simulink model "sm_trackV_lib_belt_lower_frame_s45i2u0l3_ptcld"  (R2026b)
settings: Solver=VariableStepAuto
undefined symbols (not defined in the file): Fixed, Left, Trac, track_seg_tgts_seg45i2u0r3, X, Y, Z
libraries: sm_trackV_lib_belt_contact x2, sm_lib x2, sm_trackV_lib_belt_track_s45 x1, sm_trackV_lib_belt_underc_idlerArm_i2u0l3 x1
settings Model: Creator=smiller  LastModifiedBy=smiller

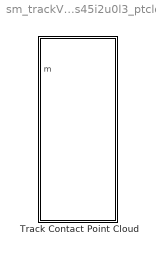
== system sm_trackV_lib_belt_lower_frame_s45i2u0l3_ptcld ==
  Track Contact Point Cloud : Subsystem  VariantControl=BeltPts  mask(Lower Frame Belted Track, Two Idler, Point Cloud){sprk_wid_roll=Trac.Sprocket.Roller.wid, sprk_rad_roll=Trac.Sprocket.Roller.rad, sprk_clr=Trac.Sprocket.Roller.clr, sprk_opc=Trac.Sprocket.Roller.opc, sprk_rad_pitch=Trac.Sprocket.Spoke.pitch_rad, sprk_spoke_rad=Trac.Sprocket.Spoke.rad, sprk_spoke_num=Trac.Sprocket.nSpokes, sprk_spoke_len=Trac.Sprocket.Spoke.len, sprk_rim_spoke_xc=Trac.Sprocket.Rim.spoke_xc, sprk_rim_ir=Trac.Sprocket.Rim.rad_inner, sprk_rim_thk=Trac.Sprocket.Rim.thk, sprk_contgeo_roller_clr=Trac.Sprocket.roller_contact.clr, sprk_contgeo_roller_opc=Trac.Sprocket.roller_contact.opc, sprk_contgeo_spoke_clr=Trac.Sprocket.spoke_contact.clr, sprk_contgeo_spoke_opc=Trac.Sprocket.spoke_contact.opc, idlerR_rad=Trac.IdlerR.rad, idlerF_rad=Trac.IdlerF.rad, idlerR_len=Trac.IdlerR.len, idlerF_len=Trac.IdlerF.len, idlerR_wheel_clr=Trac.IdlerR.Wheel.clr, idlerF_wheel_clr=Trac.IdlerF.Wheel.clr, idlerR_rim_rad=Trac.IdlerR.Rim.rad, idlerF_rim_rad=Trac.IdlerF.Rim.rad, idlerR_rim_hub_rad=Trac.IdlerR.Rim.hub_rad, idlerF_rim_hub_rad=Trac.IdlerF.Rim.hub_rad, idlerR_rim_xc=Trac.IdlerR.Rim.rim_xc, idlerF_rim_xc=Trac.IdlerF.Rim.rim_xc, idlerR_rho=Trac.IdlerR.rho, idlerF_rho=Trac.IdlerF.rho, idlerR_clr=Trac.IdlerR.clr, idlerF_clr=Trac.IdlerF.clr, idlerR_opc=Trac.IdlerR.opc, idlerF_opc=Trac.IdlerF.opc, idlerR_axle_rad=Trac.IdlerR.Axle.rad, idlerF_axle_rad=Trac.IdlerF.Axle.rad, idlerR_axle_len=Trac.IdlerR.Axle.len, idlerF_axle_len=Trac.IdlerF.Axle.len, idlerR_axle_rho=Trac.IdlerR.Axle.rho, idlerF_axle_rho=Trac.IdlerF.Axle.rho, idlerR_axle_clr=Trac.IdlerR.Axle.clr, idlerF_axle_clr=Trac.IdlerF.Axle.clr, idlerR_axle_opc=Trac.IdlerR.Axle.opc, idlerF_axle_opc=Trac.IdlerF.Axle.opc, idlerR_contgeo_clr=Trac.IdlerR.belt_contact.clr, idlerF_contgeo_clr=Trac.IdlerF.belt_contact.clr, idlerR_contgeo_opc=Trac.IdlerR.belt_contact.opc, idlerF_contgeo_opc=Trac.IdlerF.belt_contact.opc, arm_idlerc=Trac.IdlerArm.Pivot_to_Idler, arm_tens_x=Trac.IdlerArm.Pivot_to_TensionerX, arm_tens_y=Trac.IdlerArm.Pivot_to_TensionerY, arm_wid=Trac.IdlerArm.wid, arm_thk=Trac.IdlerArm.thk, arm_rho=Trac.IdlerArm.rho, arm_clr=Trac.IdlerArm.clr, arm_opc=Trac.IdlerArm.opc, roller_lower_rad=Trac.Roller.Lower.rad, roller_lower_len=Trac.Roller.Lower.len, roller_lower_rho=Trac.Roller.Lower.rho, roller_lower_clr=Trac.Roller.Lower.clr, roller_lower_opc=Trac.Roller.Lower.opc, roller_lower_rim_thk=Trac.Roller.Lower.rim_thk, roller_lower_rim_len=Trac.Roller.Lower.rim_len, roller_lower_axle_rad=Trac.Roller.Lower.Axle.rad, roller_lower_axle_len=Trac.Roller.Lower.Axle.len, roller_lower_axle_rho=Trac.Roller.Lower.Axle.rho, roller_lower_axle_clr=Trac.Roller.Lower.Axle.clr, roller_lower_axle_opc=Trac.Roller.Lower.Axle.opc, roller_lower_contgeo_clr=Trac.Roller.Lower.belt_contact.clr, roller_lower_contgeo_opc=Trac.Roller.Lower.belt_contact.opc, tensioner_cyl_len=Trac.IdlerF.Tensioner.cyl.len, tensioner_cyl_rad=Trac.IdlerF.Tensioner.cyl.rad, tensioner_cyl_rho=Trac.IdlerF.Tensioner.cyl.rho, tensioner_cyl_clr=Trac.IdlerF.Tensioner.cyl.clr, tensioner_cyl_opc=Trac.IdlerF.Tensioner.cyl.opc, tensioner_pist_len=Trac.IdlerF.Tensioner.piston.len, tensioner_pist_rad=Trac.IdlerF.Tensioner.piston.rad, tensioner_pist_rho=Trac.IdlerF.Tensioner.piston.rho, tensioner_pist_clr=Trac.IdlerF.Tensioner.piston.clr, tensioner_pist_opc=Trac.IdlerF.Tensioner.piston.opc, tensioner_br_len=Trac.IdlerF.Tensioner.bracket.len, tensioner_br_width=Trac.IdlerF.Tensioner.bracket.wid, tensioner_br_height=Trac.IdlerF.Tensioner.bracket.height, tensioner_br_thk=Trac.IdlerF.Tensioner.bracket.thk, tensioner_br_rho=Trac.IdlerF.Tensioner.bracket.rho, tensioner_br_clr=Trac.IdlerF.Tensioner.bracket.clr, tensioner_br_opc=Trac.IdlerF.Tensioner.bracket.opc, tensioner_eqpos=Trac.IdlerF.Tensioner.xeq, tensioner_x0=Trac.IdlerF.Tensioner.x0, tensioner_k=Trac.IdlerF.Tensioner.K, tensioner_b=Trac.IdlerF.Tensioner.B, popup_leftOrRight=Left, popup_trackFrame=Fixed, roller_lower_x=Trac.Frame.SprkOffLon.Lower, idlerFix_x=Trac.Frame.SprkOffLon.IdlerR, idlerArm_x=Trac.Frame.SprkOffLon.IdlerArm, tensionC_x=Trac.Frame.SprkOffLon.TensionC, frame_pivot_x=Trac.Frame.SprkOffLon.PivotFra, axle_x=Trac.Frame.SprkOffLon.Axle, roller_lower_y=Trac.Frame.SprkOffVer.Lower, idlerFix_y=Trac.Frame.SprkOffVer.IdlerR, tensionC_y=Trac.Frame.SprkOffVer.TensionC, frame_pivot_y=Trac.Frame.SprkOffVer.PivotFra, axle_y=Trac.Frame.SprkOffVer.Axle, idlerArm_y=Trac.Frame.SprkOffVer.IdlerArm, frame_mass=Trac.Frame.TrackFrame.Mass, frame_cg_offset=Trac.Frame.TrackFrame.CG, frame_moi=Trac.Frame.TrackFrame.MOI, frame_poi=Trac.Frame.TrackFrame.POI, frame_roller_cg_offset=Trac.Frame.SprkFrame.CG, frame_roller_mass=Trac.Frame.SprkFrame.Mass, frame_roller_moi=Trac.Frame.SprkFrame.MOI, frame_roller_poi=Trac.Frame.SprkFrame.POI, frame_susp_offset=Trac.Frame.SuspOffset, roller_frame_pivot_range=Trac.Frame.PivotFra.Range, roller_frame_pivot_k=Trac.Frame.PivotFra.LimitK, roller_frame_pivot_b=Trac.Frame.PivotFra.LimitB, roller_frame_pivot_tw=Trac.Frame.PivotFra.LimitTW, carc_len=Trac.Belt.l, carc_wid=Trac.Belt.w, carc_thk=Trac.Belt.pad_h, carc_mass=Trac.Belt.mass, carc_cg=Trac.Belt.cg, carc_moi=Trac.Belt.moi, carc_poi=Trac.Belt.poi, carc_clr=Trac.Belt.clr, carc_opc=Trac.Belt.opc, lug_hei=Trac.Belt.Lug.h, lug_lb=Trac.Belt.Lug.lb, lug_lt=Trac.Belt.Lug.lt, lug_w=Trac.Belt.Lug.w, lug_xc=Trac.Belt.Lug.xc, lug_clr=Trac.Belt.clr, lug_opc=Trac.Belt.opc, jointTargets=track_seg_tgts_seg45i2u0r3, trackDamping=Trac.Belt.damping, lug_line_clr=Trac.Belt.lug_contact.clr, lug_line_opc=Trac.Belt.lug_contact.opc, carc_line_clr=Trac.Belt.carcass_contact.clr, carc_line_opc=Trac.Belt.carcass_contact.opc, ptcld_belt=Trac.Belt.ground_contact.ptcld.pts, ptcld_belt_rad=Trac.Belt.ground_contact.ptcld.rad, ptcld_belt_clr=Trac.Belt.ground_contact.ptcld.clr, ptcld_belt_opc=Trac.Belt.ground_contact.ptcld.opc, K_SprocketLug=Trac.Contact.SprocketLug.K, B_SprocketLug=Trac.Contact.SprocketLug.B, TW_SprocketLug=Trac.Contact.SprocketLug.TW, K_SprocketRoller=Trac.Contact.SprocketRoller.K, B_SprocketRoller=Trac.Contact.SprocketRoller.B, TW_SprocketRoller=Trac.Contact.SprocketRoller.TW, K_IdlerFix=Trac.Contact.IdlerR.K, B_IdlerFix=Trac.Contact.IdlerR.B, TW_IdlerFix=Trac.Contact.IdlerR.TW, K_IdlerArm=Trac.Contact.IdlerF.K, B_IdlerArm=Trac.Contact.IdlerF.B, TW_IdlerArm=Trac.Contact.IdlerF.TW, K_Roller=Trac.Contact.Roller.K, B_Roller=Trac.Contact.Roller.B, TW_Roller=Trac.Contact.Roller.TW, popup_sense_roller=Actuator Torque}
      mask prompts: sprk_wid_roll "Roller Width (m)"; sprk_rad_roll "Rolling Radius (m)"; sprk_clr "Color [R G B] (0-1)"; sprk_opc "Opacity (0-1)"; sprk_rad_pitch "Pitch Radius (m)"; sprk_spoke_rad "Radius (m)"; sprk_spoke_num "Number of Spokes"; sprk_spoke_len "Length (m)"; sprk_rim_spoke_xc "Spoke Cross Section [x y] (m)"; sprk_rim_ir "Inner Radius (m)"; sprk_rim_thk "Thickness (m)"; sprk_contgeo_roller_clr "Roller Color [R G B] (0-1)"; sprk_contgeo_roller_opc "Roller Opacity (0-1)"; sprk_contgeo_spoke_clr "Spoke Color [R G B] (0-1)"; sprk_contgeo_spoke_opc "Spoke Opacity (0-1)"; arm_idlerc "Offset Pivot to Idler Center (m)"; arm_tens_x "Offset Pivot to Tensioner Long. (m)"; arm_tens_y "Offset Pivot to Tensioner Vert. (m)"; arm_wid "Idler Arm Width (m)"; arm_thk "Idler Arm Thickness (m)"; arm_rho "Idler Arm Density"; arm_clr "Idler Arm Color [R G B] (m) (0-1)"; arm_opc "Opacity (0-1)"; roller_lower_rad "Radius (m)"; roller_lower_len "Length (m)"; roller_lower_rho "Density (kg/m^3)"; roller_lower_clr "Color [R G B] (0-1)"; roller_lower_opc "Opacity (0-1)"; roller_lower_rim_thk "Thickness (m)"; roller_lower_rim_len "Length (m)"; roller_lower_axle_rad "Radius (m)"; roller_lower_axle_len "Length (m)"; roller_lower_axle_rho "Density (kg/m^3)"; roller_lower_axle_clr "Color [R G B] (0-1)"; roller_lower_axle_opc "Opacity (0-1)"; roller_lower_contgeo_clr "Color [R G B] (0-1)"; roller_lower_contgeo_opc "Opacity (0-1)"; tensioner_cyl_len "Length (m)"; tensioner_cyl_rad "Radius (m)"; tensioner_cyl_rho "Density (kg/m^3)"; tensioner_cyl_clr "Color [R G B] (0-1)"; tensioner_cyl_opc "Opacity (0-1)"; tensioner_pist_len "Piston Length (m)"; tensioner_pist_rad "Radius (m)"; tensioner_pist_rho "Density (kg/m^3)"; tensioner_pist_clr "Color [R G B] (0-1)"; tensioner_pist_opc "Opacity (0.1)"; tensioner_br_len "Length (m)"; tensioner_br_width "Width (m)"; tensioner_br_height "Height (m)"; tensioner_br_thk "Bracket Thickness (m)"; tensioner_br_rho "Density (kg/m^3)"; tensioner_br_clr "Color [R G B] (0-1)"; tensioner_br_opc "Opacity (0.1)"; tensioner_eqpos "Equilibrium Position (m)"; tensioner_x0 "Assembly Position (m)"; tensioner_k "Stiffness Coefficient (N/m)"; tensioner_b "Damping Coefficient (N/(m/s))"; popup_leftOrRight "Left or Right"; popup_trackFrame "Track Frame"; roller_lower_x "Lower Rollers (vector) (m)"; idlerFix_x "Idler Wheel Fixed (m)"; idlerArm_x "Idler Arm (m)"; tensionC_x "Tensioner Cylinder (m)"; frame_pivot_x "Frame Pivot (m)"; axle_x "Axle (m)"; roller_lower_y "Lower Rollers (m)"; idlerFix_y "Idler Wheel Fixed (m)"; tensionC_y "Tensioner Cylinder (m)"; frame_pivot_y "Frame Pivot (m)"; axle_y "Axle (m)"; idlerArm_y "Idler Arm (m)"; frame_mass "Mass (kg)"; frame_cg_offset "CG Offset from Sprocket [x y z] (m)"; frame_moi "Moments of Inertia [Ixx Iyy Izz] (kg*m^2)"; frame_poi "Products of Inertia [Ixx Iyy Izz] (kg*m^2)"; frame_roller_cg_offset "CG Offset from Sprocket [x y z] (m)"; frame_roller_mass "Mass (kg)"; frame_roller_moi "Moments of Inertia [Ixx Iyy Izz] (kg*m^2)"; frame_roller_poi "Products of Inertia [Ixx Iyy Izz] (kg*m^2)"; frame_susp_offset "Suspension Offset from Sprocket [x y z] (m)"; roller_frame_pivot_range "Range (deg)"; roller_frame_pivot_k "Stop stiffness (N*m/deg)"; roller_frame_pivot_b "Stop damping (N*m/(deg*sec)"; roller_frame_pivot_tw "Stop transition width (deg)"; carc_len "Length (m)"; carc_wid "Width (m)"; carc_thk "Thickness (m)"; carc_mass "Mass (kg)"; carc_cg "CG [x y z] (kg)"; carc_moi "Moments of Inertia [Ixx Iyy Izz] (kg*m^2)"; carc_poi "Products of Inertia [Iyz Ixz Ixy] (kg*m^2)"; carc_clr "Color [R G B]"; carc_opc "Opacity (0-1)"; lug_hei "Height (m)"; lug_lb "Length Base (m)"; lug_lt "Length Tip (m)"; lug_w "Width (m)"; lug_xc "Profile [x y] (m)"; lug_clr "Color [R G B]"; lug_opc "Opacity (0-1)"; jointTargets "Joint Targets (structure)"; trackDamping "Joint Damping N*m/(deg/s)"; lug_line_clr "Color [R G B] (0-1)"; lug_line_opc "Opacity (0-1)"; carc_line_clr "Color [R G B] (0-1)"; carc_line_opc "Opacity (0-1)"; ptcld_belt "Points [x y z] (m)"; ptcld_belt_rad "Radius (m)"; ptcld_belt_clr "Color [R G B] (0-1)"; ptcld_belt_opc "Opacity (0-1)"; K_SprocketLug "Normal Stiffness (N/m)"; B_SprocketLug "Normal Damping (N/(m/s))"; TW_SprocketLug "Normal Transition Width (m)"; K_SprocketRoller "Normal Stiffness (N/m)"; B_SprocketRoller "Normal Damping (N/(m/s))"; TW_SprocketRoller "Normal Transition Width (m)"; K_IdlerFix "Normal Stiffness (N/m)"; B_IdlerFix "Normal Damping (N/(m/s))"; TW_IdlerFix "Normal Transition Width (m)"; K_IdlerArm "Normal Stiffness (N/m)"; B_IdlerArm "Normal Damping (N/(m/s))"; TW_IdlerArm "Normal Transition Width (m)"; K_Roller "Normal Stiffness (N/m)"; B_Roller "Normal Damping (N/(m/s))"; TW_Roller "Normal Transition Width (m)"; popup_sense_roller "Roller"
      mask help: Models a segmented belt with undercarriage. Contact geometry (point cloud) in belt segment enables contact with the ground. Includes sprocket, rollers, and idler with tensioner. The sprocket has a 1D rotational mechanical interface to the drivetrain.
      settings: AttributesFormatString=|
      | %<popup_leftOrRight>
      | %<popup_sense_roller>
      | %<popup_trackFrame>
      mask TypeOptions sprk_wid_roll: Undercarriage/sprk_wid_roll
      mask TypeOptions sprk_rad_roll: Undercarriage/sprk_rad_roll
      mask TypeOptions sprk_clr: Undercarriage/sprk_clr
      mask TypeOptions sprk_opc: Undercarriage/sprk_opc
      mask TypeOptions sprk_rad_pitch: Undercarriage/sprk_rad_pitch
      mask TypeOptions sprk_spoke_rad: Undercarriage/sprk_spoke_rad
      mask TypeOptions sprk_spoke_num: Undercarriage/sprk_spoke_num
      mask TypeOptions sprk_spoke_len: Undercarriage/sprk_spoke_len
      mask TypeOptions sprk_rim_spoke_xc: Undercarriage/sprk_rim_spoke_xc
      mask TypeOptions sprk_rim_ir: Undercarriage/sprk_rim_ir
      mask TypeOptions sprk_rim_thk: Undercarriage/sprk_rim_thk
      mask TypeOptions sprk_contgeo_roller_clr: Undercarriage/sprk_contgeo_roller_clr
      mask TypeOptions sprk_contgeo_roller_opc: Undercarriage/sprk_contgeo_roller_opc
      mask TypeOptions sprk_contgeo_spoke_clr: Undercarriage/sprk_contgeo_spoke_clr
      mask TypeOptions sprk_contgeo_spoke_opc: Undercarriage/sprk_contgeo_spoke_opc
      mask TypeOptions idlerR_rad: Undercarriage/idlerR_rad
      mask TypeOptions idlerF_rad: Undercarriage/idlerF_rad
      mask TypeOptions idlerR_len: Undercarriage/idlerR_len
      mask TypeOptions idlerF_len: Undercarriage/idlerF_len
      mask TypeOptions idlerR_wheel_clr: Undercarriage/idlerR_wheel_clr
      mask TypeOptions idlerF_wheel_clr: Undercarriage/idlerF_wheel_clr
      mask TypeOptions idlerR_rim_rad: Undercarriage/idlerR_rim_rad
      mask TypeOptions idlerF_rim_rad: Undercarriage/idlerF_rim_rad
      mask TypeOptions idlerR_rim_hub_rad: Undercarriage/idlerR_rim_hub_rad
      mask TypeOptions idlerF_rim_hub_rad: Undercarriage/idlerF_rim_hub_rad
      mask TypeOptions idlerR_rim_xc: Undercarriage/idlerR_rim_xc
      mask TypeOptions idlerF_rim_xc: Undercarriage/idlerF_rim_xc
      mask TypeOptions idlerR_rho: Undercarriage/idlerR_rho
      mask TypeOptions idlerF_rho: Undercarriage/idlerF_rho
      mask TypeOptions idlerR_clr: Undercarriage/idlerR_clr
      mask TypeOptions idlerF_clr: Undercarriage/idlerF_clr
      mask TypeOptions idlerR_opc: Undercarriage/idlerR_opc
      mask TypeOptions idlerF_opc: Undercarriage/idlerF_opc
      mask TypeOptions idlerR_axle_rad: Undercarriage/idlerR_axle_rad
      mask TypeOptions idlerF_axle_rad: Undercarriage/idlerF_axle_rad
      mask TypeOptions idlerR_axle_len: Undercarriage/idlerR_axle_len
      mask TypeOptions idlerF_axle_len: Undercarriage/idlerF_axle_len
      mask TypeOptions idlerR_axle_rho: Undercarriage/idlerR_axle_rho
      mask TypeOptions idlerF_axle_rho: Undercarriage/idlerF_axle_rho
      mask TypeOptions idlerR_axle_clr: Undercarriage/idlerR_axle_clr
      mask TypeOptions idlerF_axle_clr: Undercarriage/idlerF_axle_clr
      mask TypeOptions idlerR_axle_opc: Undercarriage/idlerR_axle_opc
      mask TypeOptions idlerF_axle_opc: Undercarriage/idlerF_axle_opc
      mask TypeOptions idlerR_contgeo_clr: Undercarriage/idlerR_contgeo_clr
      mask TypeOptions idlerF_contgeo_clr: Undercarriage/idlerF_contgeo_clr
      mask TypeOptions idlerR_contgeo_opc: Undercarriage/idlerR_contgeo_opc
      mask TypeOptions idlerF_contgeo_opc: Undercarriage/idlerF_contgeo_opc
      mask TypeOptions arm_idlerc: Undercarriage/arm_idlerc
      mask TypeOptions arm_tens_x: Undercarriage/arm_tens_x
      mask TypeOptions arm_tens_y: Undercarriage/arm_tens_y
      mask TypeOptions arm_wid: Undercarriage/arm_wid
      mask TypeOptions arm_thk: Undercarriage/arm_thk
      mask TypeOptions arm_rho: Undercarriage/arm_rho
      mask TypeOptions arm_clr: Undercarriage/arm_clr
      mask TypeOptions arm_opc: Undercarriage/arm_opc
      mask TypeOptions roller_lower_rad: Undercarriage/roller_lower_rad
      mask TypeOptions roller_lower_len: Undercarriage/roller_lower_len
      mask TypeOptions roller_lower_rho: Undercarriage/roller_lower_rho
      mask TypeOptions roller_lower_clr: Undercarriage/roller_lower_clr
      mask TypeOptions roller_lower_opc: Undercarriage/roller_lower_opc
      mask TypeOptions roller_lower_rim_thk: Undercarriage/roller_lower_rim_thk
      mask TypeOptions roller_lower_rim_len: Undercarriage/roller_lower_rim_len
      mask TypeOptions roller_lower_axle_rad: Undercarriage/roller_lower_axle_rad
      mask TypeOptions roller_lower_axle_len: Undercarriage/roller_lower_axle_len
      mask TypeOptions roller_lower_axle_rho: Undercarriage/roller_lower_axle_rho
      mask TypeOptions roller_lower_axle_clr: Undercarriage/roller_lower_axle_clr
      mask TypeOptions roller_lower_axle_opc: Undercarriage/roller_lower_axle_opc
      mask TypeOptions roller_lower_contgeo_clr: Undercarriage/roller_lower_contgeo_clr
      mask TypeOptions roller_lower_contgeo_opc: Undercarriage/roller_lower_contgeo_opc
      mask TypeOptions tensioner_cyl_len: Undercarriage/tensioner_cyl_len
      mask TypeOptions tensioner_cyl_rad: Undercarriage/tensioner_cyl_rad
      mask TypeOptions tensioner_cyl_rho: Undercarriage/tensioner_cyl_rho
      mask TypeOptions tensioner_cyl_clr: Undercarriage/tensioner_cyl_clr
      mask TypeOptions tensioner_cyl_opc: Undercarriage/tensioner_cyl_opc
      mask TypeOptions tensioner_pist_len: Undercarriage/tensioner_pist_len
      mask TypeOptions tensioner_pist_rad: Undercarriage/tensioner_pist_rad
      mask TypeOptions tensioner_pist_rho: Undercarriage/tensioner_pist_rho
      mask TypeOptions tensioner_pist_clr: Undercarriage/tensioner_pist_clr
      mask TypeOptions tensioner_pist_opc: Undercarriage/tensioner_pist_opc
      mask TypeOptions tensioner_br_len: Undercarriage/tensioner_br_len
      mask TypeOptions tensioner_br_width: Undercarriage/tensioner_br_width
      mask TypeOptions tensioner_br_height: Undercarriage/tensioner_br_height
      mask TypeOptions tensioner_br_thk: Undercarriage/tensioner_br_thk
      mask TypeOptions tensioner_br_rho: Undercarriage/tensioner_br_rho
      mask TypeOptions tensioner_br_clr: Undercarriage/tensioner_br_clr
      mask TypeOptions tensioner_br_opc: Undercarriage/tensioner_br_opc
      mask TypeOptions tensioner_eqpos: Undercarriage/tensioner_eqpos
      mask TypeOptions tensioner_x0: Undercarriage/tensioner_x0
      mask TypeOptions tensioner_k: Undercarriage/tensioner_k
      mask TypeOptions tensioner_b: Undercarriage/tensioner_b
      mask TypeOptions popup_leftOrRight: Undercarriage/popup_leftOrRight
      mask TypeOptions popup_trackFrame: Undercarriage/popup_trackFrame
      mask TypeOptions roller_lower_x: Undercarriage/roller_lower_x
      mask TypeOptions idlerFix_x: Undercarriage/idlerFix_x
      mask TypeOptions idlerArm_x: Undercarriage/idlerArm_x
      mask TypeOptions tensionC_x: Undercarriage/tensionC_x
      mask TypeOptions frame_pivot_x: Undercarriage/frame_pivot_x
      mask TypeOptions axle_x: Undercarriage/axle_x
      mask TypeOptions roller_lower_y: Undercarriage/roller_lower_y
      mask TypeOptions idlerFix_y: Undercarriage/idlerFix_y
      mask TypeOptions tensionC_y: Undercarriage/tensionC_y
      mask TypeOptions frame_pivot_y: Undercarriage/frame_pivot_y
      mask TypeOptions axle_y: Undercarriage/axle_y
      mask TypeOptions idlerArm_y: Undercarriage/idlerArm_y
      mask TypeOptions frame_mass: Undercarriage/frame_mass
      mask TypeOptions frame_cg_offset: Undercarriage/frame_cg_offset
      mask TypeOptions frame_moi: Undercarriage/frame_moi
      mask TypeOptions frame_poi: Undercarriage/frame_poi
      mask TypeOptions frame_roller_cg_offset: Undercarriage/frame_roller_cg_offset
      mask TypeOptions frame_roller_mass: Undercarriage/frame_roller_mass
      mask TypeOptions frame_roller_moi: Undercarriage/frame_roller_moi
      mask TypeOptions frame_roller_poi: Undercarriage/frame_roller_poi
      mask TypeOptions frame_susp_offset: Undercarriage/frame_susp_offset
      mask TypeOptions roller_frame_pivot_range: Undercarriage/roller_frame_pivot_range
      mask TypeOptions roller_frame_pivot_k: Undercarriage/roller_frame_pivot_k
      mask TypeOptions roller_frame_pivot_b: Undercarriage/roller_frame_pivot_b
      mask TypeOptions roller_frame_pivot_tw: Undercarriage/roller_frame_pivot_tw
      mask TypeOptions carc_len: Track/carc_len
      mask TypeOptions carc_wid: Track/carc_wid
      mask TypeOptions carc_thk: Track/carc_thk
      mask TypeOptions carc_mass: Track/carc_mass
      mask TypeOptions carc_cg: Track/carc_cg
      mask TypeOptions carc_moi: Track/carc_moi
      mask TypeOptions carc_poi: Track/carc_poi
      mask TypeOptions carc_clr: Track/carc_clr
      mask TypeOptions carc_opc: Track/carc_opc
      mask TypeOptions lug_hei: Track/lug_hei
      mask TypeOptions lug_lb: Track/lug_lb
      mask TypeOptions lug_lt: Track/lug_lt
      mask TypeOptions lug_w: Track/lug_w
      mask TypeOptions lug_xc: Track/lug_xc
      mask TypeOptions lug_clr: Track/lug_clr
      mask TypeOptions lug_opc: Track/lug_opc
      mask TypeOptions jointTargets: Track/jointTargets
      mask TypeOptions trackDamping: Track/trackDamping
      mask TypeOptions lug_line_clr: Track/lug_line_clr
      mask TypeOptions lug_line_opc: Track/lug_line_opc
      mask TypeOptions carc_line_clr: Track/carc_line_clr
      mask TypeOptions carc_line_opc: Track/carc_line_opc
      mask TypeOptions ptcld_belt: Track/ptcld_belt
      mask TypeOptions ptcld_belt_rad: Track/ptcld_belt_rad
      mask TypeOptions ptcld_belt_clr: Track/ptcld_belt_clr
      mask TypeOptions ptcld_belt_opc: Track/ptcld_belt_opc
      mask TypeOptions K_SprocketLug:
      | CF
      | Sprocket
      | Lugs/K_SprocketLug
      mask TypeOptions B_SprocketLug:
      | CF
      | Sprocket
      | Lugs/B_SprocketLug
      mask TypeOptions TW_SprocketLug:
      | CF
      | Sprocket
      | Lugs/TW_SprocketLug
      mask TypeOptions K_SprocketRoller:
      | CF
      | Belt
      | Roller/K_SprocketRoller
      mask TypeOptions B_SprocketRoller:
      | CF
      | Belt
      | Roller/B_SprocketRoller
      mask TypeOptions TW_SprocketRoller:
      | CF
      | Belt
      | Roller/TW_SprocketRoller
      mask TypeOptions K_IdlerFix:
      | CF
      | Belt
      | Roller/K_IdlerFix
      mask TypeOptions B_IdlerFix:
      | CF
      | Belt
      | Roller/B_IdlerFix
      mask TypeOptions TW_IdlerFix:
      | CF
      | Belt
      | Roller/TW_IdlerFix
      mask TypeOptions K_IdlerArm:
      | CF
      | Belt
      | Roller/K_IdlerArm
      mask TypeOptions B_IdlerArm:
      | CF
      | Belt
      | Roller/B_IdlerArm
      mask TypeOptions TW_IdlerArm:
      | CF
      | Belt
      | Roller/TW_IdlerArm
      mask TypeOptions K_Roller:
      | CF
      | Belt
      | Roller/K_Roller
      mask TypeOptions B_Roller:
      | CF
      | Belt
      | Roller/B_Roller
      mask TypeOptions TW_Roller:
      | CF
      | Belt
      | Roller/TW_Roller
      mask TypeOptions popup_sense_roller: Undercarriage/popup_sense_roller
      mask DialogControl cont_sprocket Prompt: Sprocket
      mask DialogControl cont_sprk_roller Prompt: Roller
      mask DialogControl cont_sprk_spoke Prompt: Spoke
      mask DialogControl cont_sprk_rim Prompt: Rim
      mask DialogControl cont_contgeo_sprk Prompt: Contact Geometry
      mask DialogControl cont_idler Prompt: Idler
      mask DialogControl cont_idler_roller Prompt: Roller
      mask DialogControl text_idler_rear Prompt: Rear
      mask DialogControl text_idler_front Prompt: Front
      mask DialogControl text_idler_rad Prompt: Radius (m)
      mask DialogControl text_idler_len Prompt: Length (m)
      mask DialogControl text_idler_wheel_clr Prompt: Wheel Color [R G B] (0-1)
      mask DialogControl cont_idler_rim Prompt: Rim
      mask DialogControl text_idler_rim_rad Prompt: Radius (m)
      mask DialogControl text_idler_hub_rad Prompt: Hub Radius (m)
      mask DialogControl text_idler_rim_xc Prompt: Cross Section [x y] (m)
      mask DialogControl text_idler_rho Prompt: Density (kg/m^3)
      mask DialogControl text_idler_clr Prompt: Color [R G B] (0-1)
      mask DialogControl text_idler_opc Prompt: Opacity (0-1)
      mask DialogControl cont_idler_axle Prompt: Axle
      mask DialogControl text_idler_axle_rad Prompt: Radius (m)
      mask DialogControl text_idler_axle_len Prompt: Length (m)
      mask DialogControl text_idler_axle_rho Prompt: Density (kg/m^3)
      mask DialogControl text_idler_axle_clr Prompt: Color [R G B] (0-1)
      mask DialogControl text_idler_axle_opc Prompt: Opacity (0-1)
      mask DialogControl cont_idler_pin_contgeo Prompt: Contact Geometry
      mask DialogControl text_idler_contgeo_clr Prompt: Color [R G B] (0-1)
      mask DialogControl text_idler_contgeo_opc Prompt: Opacity (0-1)
      mask DialogControl cont_idler_arm Prompt: Idler Arm
      mask DialogControl cont_roller_lower Prompt: Rollers
      mask DialogControl cont_rollerL_roller Prompt: Roller
      mask DialogControl cont_rollerL_rim Prompt: Rim
      mask DialogControl cont_rollerL_axle Prompt: Axle
      mask DialogControl cont_rollerL_contgeo Prompt: Contact Geometry
      mask DialogControl cont_tensioner Prompt: Tensioner
      mask DialogControl cont_tens_cyl Prompt: Cylinder
      mask DialogControl cont_tens_pist Prompt: Piston
      mask DialogControl cont_tens_brk Prompt: Bracket
      mask DialogControl cont_tens_asy Prompt: Assembly
      mask DialogControl cont_frame Prompt: Frame
      mask DialogControl cont_frame_lon Prompt: Longitudinal Offsets from Sprocket
      mask DialogControl cont_frame_ver Prompt: Vertical Offsets from Sprocket
      mask DialogControl cont_frame_mass Prompt: Mass and Inertia
      mask DialogControl cont_sprocket_frame Prompt: Sprocket Frame
      mask DialogControl cont_roller_frame Prompt: Roller Frame
      mask DialogControl cont_susp_offset Prompt: Suspension Offsets
      mask DialogControl cont_frame_pivot Prompt: Frame Pivot
      mask DialogControl cont_belt Prompt: Belt
      mask DialogControl cont_carcass Prompt: Carcass
      mask DialogControl cont_lug Prompt: Lug
      mask DialogControl cont_belt_assy Prompt: Assembly
      mask DialogControl cont_contgeo_belt Prompt: Contact Geometry
      mask DialogControl cont_contgeo_lug2sprk Prompt: Sprocket to Lug
      mask DialogControl cont_contgeo_carc2roll Prompt: Carcass to Rollers
      mask DialogControl cont_contgeo_carc2gnd Prompt: Carcass to Ground
      mask DialogControl cont_contact Prompt: Contact
      mask DialogControl cont_contact_lug2sprk Prompt: Lug to Sprocket
      mask DialogControl cont_contact_carc2sprk Prompt: Carcass to Sprocket Roller
      mask DialogControl cont_contact_carc2idlerX Prompt: Carcass to Fixed Idler
      mask DialogControl cont_contact_carc2idlerA Prompt: Carcass to Moving Idler
      mask DialogControl cont_contact_carc2roller Prompt: Carcass to Rollers
      mask DialogControl cont_sensing Prompt: Sensing
      mask Display: image('sm_belt_track_2i_ptcld_topview_IMAGE.png')

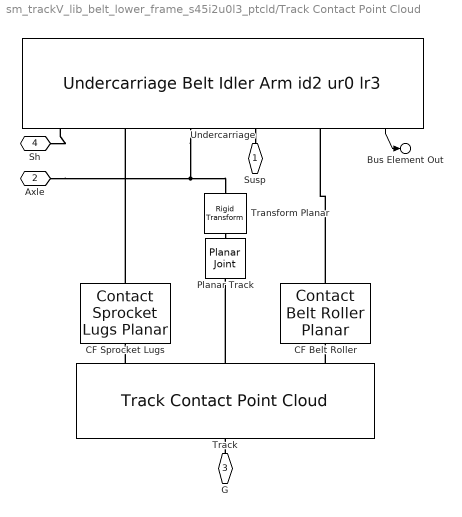
== system sm_trackV_lib_belt_lower_frame_s45i2u0l3_ptcld/Track Contact Point Cloud ==
  " CF Sprocket Lugs" : sm_trackV_lib_belt_contact/Contact Sprocket Lugs Planar  K_SprocketLug=K_SprocketLug  B_SprocketLug=B_SprocketLug  TW_SprocketLug=TW_SprocketLug
  CF Belt Roller : sm_trackV_lib_belt_contact/Contact Belt Roller Planar  K_SprocketRoller=K_SprocketRoller  B_SprocketRoller=B_SprocketRoller  TW_SprocketRoller=TW_SprocketRoller  K_IdlerFix=K_IdlerFix  B_IdlerFix=B_IdlerFix  TW_IdlerFix=TW_IdlerFix  K_IdlerArm=K_IdlerArm  B_IdlerArm=B_IdlerArm  TW_IdlerArm=TW_IdlerArm  K_Roller=K_Roller  B_Roller=B_Roller  TW_Roller=TW_Roller
  Planar Track : sm_lib/Joints/Planar Joint  JointMode=Normal  CompositeWrenchDir=FollowerOnBase  CompositeWrenchFrame=BaseFrame  SenseConstraintForce=off  SenseConstraintTorque=off  SenseTotalForce=off  SenseTotalTorque=off  PxPositionTargetSpecify=on  PxPositionTargetPriority=High  PxPositionTargetValue=0  PxPositionTargetValueUnits=m  PxVelocityTargetSpecify=off  PxVelocityTargetPriority=High  PxVelocityTargetValue=0  PxVelocityTargetValueUnits=m/s  PxEquilibriumPosition=0  PxEquilibriumPositionUnits=m  PxSpringStiffness=0  PxSpringStiffnessUnits=N/m  PxDampingCoefficient=0  PxDampingCoefficientUnits=N/(m/s)  PxLowerLimitSpecify=off  PxLowerLimitBound=-1  PxLowerLimitBoundUnits=m  PxLowerLimitStiffness=1e6  PxLowerLimitStiffnessUnits=N/m  PxLowerLimitDamping=1e3  PxLowerLimitDampingUnits=N/(m/s)  PxLowerLimitTransitionRegionWidth=1e-4  PxLowerLimitTransitionRegionWidthUnits=m  PxUpperLimitSpecify=off  PxUpperLimitBound=1  PxUpperLimitBoundUnits=m  PxUpperLimitStiffness=1e6  PxUpperLimitStiffnessUnits=N/m  PxUpperLimitDamping=1e3  PxUpperLimitDampingUnits=N/(m/s)  PxUpperLimitTransitionRegionWidth=1e-4  PxUpperLimitTransitionRegionWidthUnits=m  PxTorqueActuationMode=NoTorque  PxMotionActuationMode=ComputedMotion  PxSensePosition=off  PxSenseVelocity=off  PxSenseAcceleration=off  PxSenseTorqueForce=off  PxSenseLowerLimitTorqueForce=off  PxSenseUpperLimitTorqueForce=off  PyPositionTargetSpecify=on  PyPositionTargetPriority=High  PyPositionTargetValue=0  PyPositionTargetValueUnits=m  PyVelocityTargetSpecify=off  PyVelocityTargetPriority=High  PyVelocityTargetValue=0  PyVelocityTargetValueUnits=m/s  PyEquilibriumPosition=0  PyEquilibriumPositionUnits=m  PySpringStiffness=0  PySpringStiffnessUnits=N/m  PyDampingCoefficient=0  PyDampingCoefficientUnits=N/(m/s)  PyLowerLimitSpecify=off  PyLowerLimitBound=-1  PyLowerLimitBoundUnits=m  PyLowerLimitStiffness=1e6  PyLowerLimitStiffnessUnits=N/m  PyLowerLimitDamping=1e3  PyLowerLimitDampingUnits=N/(m/s)  PyLowerLimitTransitionRegionWidth=1e-4  PyLowerLimitTransitionRegionWidthUnits=m  PyUpperLimitSpecify=off  PyUpperLimitBound=1  PyUpperLimitBoundUnits=m  PyUpperLimitStiffness=1e6  PyUpperLimitStiffnessUnits=N/m  PyUpperLimitDamping=1e3  PyUpperLimitDampingUnits=N/(m/s)  PyUpperLimitTransitionRegionWidth=1e-4  PyUpperLimitTransitionRegionWidthUnits=m  PyTorqueActuationMode=NoTorque  PyMotionActuationMode=ComputedMotion  PySensePosition=off  PySenseVelocity=off  PySenseAcceleration=off  PySenseTorqueForce=off  PySenseLowerLimitTorqueForce=off  PySenseUpperLimitTorqueForce=off  RzPositionTargetSpecify=off  RzPositionTargetPriority=High  RzPositionTargetValue=0  RzPositionTargetValueUnits=deg  RzVelocityTargetSpecify=off  RzVelocityTargetPriority=High  RzVelocityTargetValue=0  RzVelocityTargetValueUnits=deg/s  RzEquilibriumPosition=0  RzEquilibriumPositionUnits=deg  RzSpringStiffness=0  RzSpringStiffnessUnits=N*m/deg  RzDampingCoefficient=0  RzDampingCoefficientUnits=N*m/(deg/s)  RzLowerLimitSpecify=off  RzLowerLimitBound=-90  RzLowerLimitBoundUnits=deg  RzLowerLimitStiffness=1e4  RzLowerLimitStiffnessUnits=N*m/deg  RzLowerLimitDamping=10  RzLowerLimitDampingUnits=N*m/(deg/s)  RzLowerLimitTransitionRegionWidth=0.1  RzLowerLimitTransitionRegionWidthUnits=deg  RzUpperLimitSpecify=off  RzUpperLimitBound=90  RzUpperLimitBoundUnits=deg  RzUpperLimitStiffness=1e4  RzUpperLimitStiffnessUnits=N*m/deg  RzUpperLimitDamping=10  RzUpperLimitDampingUnits=N*m/(deg/s)  RzUpperLimitTransitionRegionWidth=0.1  RzUpperLimitTransitionRegionWidthUnits=deg  RzTorqueActuationMode=NoTorque  RzMotionActuationMode=ComputedMotion  RzSensePosition=off  RzSenseVelocity=off  RzSenseAcceleration=off  RzSenseTorqueForce=off  RzSenseLowerLimitTorqueForce=off  RzSenseUpperLimitTorqueForce=off
  Track : sm_trackV_lib_belt_track_s45/Track Contact Point Cloud  carc_len=carc_len  carc_wid=carc_wid  carc_thk=carc_thk  carc_mass=carc_mass  carc_cg=carc_cg  carc_moi=carc_moi  carc_poi=carc_poi  carc_clr=carc_clr  carc_opc=carc_opc  lug_hei=lug_hei  lug_lb=lug_lb  lug_lt=lug_lt  lug_w=lug_w  lug_xc=lug_xc  lug_clr=lug_clr  lug_opc=lug_opc  jointTargets=jointTargets  trackDamping=trackDamping  lug_line_clr=lug_line_clr  lug_line_opc=lug_line_opc  carc_line_clr=carc_line_clr  carc_line_opc=carc_line_opc  ptcld_belt=ptcld_belt  ptcld_belt_rad=ptcld_belt_rad  ptcld_belt_clr=ptcld_belt_clr  ptcld_belt_opc=ptcld_belt_opc
  Transform Planar : sm_lib/Frames and Transforms/Rigid Transform  RotationMethod=StandardAxis  FollAlignAxisA=+X  BaseAlignAxisA=+Y  FollAlignAxisB=+Y  BaseAlignAxisB=+Z  RotationStandardAxis=+Z  RotationAngle=-jointTargets{1,3}/2  RotationAngleUnits=deg  RotationArbitraryAxis=[0 0 1]  RotationSequenceAxes=FollowerAxes  RotationSequence=XYX  RotationSequenceAngles=[0 0 0]  RotationSequenceAnglesUnits=deg  RotationMatrix=[1 0 0; 0 1 0; 0 0 1]  Quaternion=[1 0 0 0]  TranslationMethod=StandardAxis  TranslationCartesianOffset=[0 0 0]  TranslationCartesianOffsetUnits=m  TranslationStandardAxis=+Y  TranslationStandardOffset=-sprk_rad_roll-carc_thk/2  TranslationStandardOffsetUnits=m  TranslationROffset=0  TranslationROffsetUnits=m  TranslationThetaOffset=0  TranslationThetaOffsetUnits=deg  TranslationZOffset=0  TranslationZOffsetUnits=m
  Undercarriage : sm_trackV_lib_belt_underc_idlerArm_i2u0l3/Undercarriage Belt Idler Arm id2 ur0 lr3  popup_leftOrRight=Left  sprk_rad_roll=sprk_rad_roll  sprk_wid_roll=sprk_wid_roll  sprk_clr=sprk_clr  sprk_opc=sprk_opc  sprk_rim_ir=sprk_rim_ir  sprk_rim_thk=sprk_rim_thk  sprk_rim_spoke_xc=sprk_rim_spoke_xc  sprk_rad_pitch=sprk_rad_pitch  sprk_spoke_rad=sprk_spoke_rad  sprk_spoke_len=sprk_spoke_len  sprk_spoke_num=sprk_spoke_num  sprk_contgeo_roller_clr=sprk_contgeo_roller_clr  sprk_contgeo_roller_opc=sprk_contgeo_roller_opc  sprk_contgeo_spoke_clr=sprk_contgeo_spoke_clr  sprk_contgeo_spoke_opc=sprk_contgeo_spoke_opc  idlerR_rad=idlerR_rad  idlerF_rad=idlerF_rad  idlerR_len=idlerR_len  idlerF_len=idlerF_len  idlerR_rho=idlerR_rho  idlerF_rho=idlerF_rho  idlerR_wheel_clr=idlerR_wheel_clr  idlerF_wheel_clr=idlerF_wheel_clr  idlerR_rim_rad=idlerR_rim_rad  idlerF_rim_rad=idlerF_rim_rad  idlerR_rim_hub_rad=idlerR_rim_hub_rad  idlerF_rim_hub_rad=idlerF_rim_hub_rad  idlerR_rim_xc=idlerR_rim_xc  idlerF_rim_xc=idlerF_rim_xc  idlerR_clr=idlerR_clr  idlerF_clr=idlerF_clr  idlerR_opc=idlerR_opc  idlerF_opc=idlerF_opc  idlerR_axle_rad=idlerR_axle_rad  idlerF_axle_rad=idlerF_axle_rad  idlerR_axle_len=idlerR_axle_len  idlerF_axle_len=idlerF_axle_len  idlerR_axle_rho=idlerR_axle_rho  idlerF_axle_rho=idlerF_axle_rho  idlerR_axle_clr=idlerR_axle_clr  idlerF_axle_clr=idlerF_axle_clr  idlerR_axle_opc=idlerR_axle_opc  idlerF_axle_opc=idlerF_axle_opc  idlerR_contgeo_clr=idlerR_contgeo_clr  idlerF_contgeo_clr=idlerF_contgeo_clr  idlerR_contgeo_opc=idlerR_contgeo_opc  idlerF_contgeo_opc=idlerF_contgeo_opc  arm_idlerc=arm_idlerc  arm_tens_x=arm_tens_x  arm_tens_y=arm_tens_y  arm_wid=arm_wid  arm_thk=arm_thk  arm_rho=arm_rho  arm_clr=arm_clr  arm_opc=arm_opc  roller_lower_len=roller_lower_len  roller_lower_rad=roller_lower_rad  roller_lower_rho=roller_lower_rho  roller_lower_clr=roller_lower_clr  roller_lower_opc=roller_lower_opc  roller_lower_rim_thk=roller_lower_rim_thk  roller_lower_rim_len=roller_lower_rim_len  roller_lower_axle_len=roller_lower_axle_len  roller_lower_axle_rad=roller_lower_axle_rad  roller_lower_axle_rho=roller_lower_axle_rho  roller_lower_axle_clr=roller_lower_axle_clr  roller_lower_axle_opc=roller_lower_axle_opc  roller_lower_contgeo_clr=roller_lower_contgeo_clr  roller_lower_contgeo_opc=roller_lower_contgeo_opc  tensioner_cyl_len=tensioner_cyl_len  tensioner_cyl_rad=tensioner_cyl_rad  tensioner_cyl_rho=tensioner_cyl_rho  tensioner_cyl_clr=tensioner_cyl_clr  tensioner_cyl_opc=tensioner_cyl_opc  tensioner_pist_len=tensioner_pist_len  tensioner_pist_rad=tensioner_pist_rad  tensioner_pist_rho=tensioner_pist_rho  tensioner_pist_clr=tensioner_pist_clr  tensioner_pist_opc=tensioner_pist_opc  tensioner_br_len=tensioner_br_len  tensioner_br_width=tensioner_br_width  tensioner_br_height=tensioner_br_height  tensioner_br_thk=tensioner_br_thk  tensioner_br_rho=tensioner_br_rho  tensioner_br_clr=tensioner_br_clr  tensioner_br_opc=tensioner_br_opc  tensioner_eqpos=tensioner_eqpos  tensioner_x0=tensioner_x0  tensioner_k=tensioner_k  tensioner_b=tensioner_b  popup_trackFrame=Fixed  roller_lower_x=roller_lower_x  axle_x=axle_x  idlerFix_x=idlerFix_x  frame_pivot_x=frame_pivot_x  tensionC_x=tensionC_x  idlerArm_x=idlerArm_x  roller_lower_y=roller_lower_y  axle_y=axle_y  idlerArm_y=idlerArm_y  idlerFix_y=idlerFix_y  frame_pivot_y=frame_pivot_y  tensionC_y=tensionC_y  frame_cg_offset=frame_cg_offset  frame_mass=frame_mass  frame_moi=frame_moi  frame_poi=frame_poi  frame_roller_cg_offset=frame_roller_cg_offset  frame_roller_mass=frame_roller_mass  frame_roller_moi=frame_roller_moi  frame_roller_poi=frame_roller_poi  roller_frame_pivot_range=roller_frame_pivot_range  roller_frame_pivot_k=roller_frame_pivot_k  roller_frame_pivot_b=roller_frame_pivot_b  roller_frame_pivot_tw=roller_frame_pivot_tw  frame_susp_offset=frame_susp_offset  popup_sense_roller=Actuator Torque
  Susp : PMIOPort  Side=Left
  Axle : PMIOPort  Port=2  Side=Left
  G : PMIOPort  Port=3  Side=Right
  Sh : PMIOPort  Port=4  Side=Right
  Bus Element Out : Outport  PortName=m  Element=Underc
  wires:
  Undercarriage/1 -> Bus Element Out/1
  connections:
  Undercarriage/RConn3 -- Transform Planar/LConn1 -- Axle/RConn1
  CF Belt Roller/RConn1 -- Undercarriage/RConn1
  Transform Planar/RConn1 -- Planar Track/LConn1
  Track/RConn1 -- " CF Sprocket Lugs"/RConn1
  G/RConn1 -- Track/LConn1
  Track/RConn3 -- CF Belt Roller/LConn1
  Track/RConn2 -- Planar Track/RConn1
  " CF Sprocket Lugs"/LConn1 -- Undercarriage/RConn4
  Sh/RConn1 -- Undercarriage/RConn5
  Undercarriage/RConn2 -- Susp/RConn1
